simulink model "VIRTUAL_self_driving_stack_autoLocalize_v2"  (R2026a)
settings: Solver=ode1  StopTime=inf  FixedStep=1/500  EnableMultiTasking=on
values from neighbouring files (symbols this model uses):
  Controller_Sample_Time = 1/500    (= 0.002)    [Setup_QCar2_Params_Addons.m]
  path_x4 = [-0.614 -0.604 -0.594 -0.584 -0.574 -0.564 -0.554 -0.544 -0.534 -0.524 -0.514 -0.504 ... (1761 elements, 1761x1)]    [SDCS_Paths_7.mat]
  path_y4 = [-1.0887 -1.0887 -1.0887 -1.0887 -1.0887 -1.0887 -1.0887 -1.0887 -1.0887 -1.0887 -1.0887 -1.0887 ... (1761 elements, 1761x1)]    [SDCS_Paths_7.mat]
undefined symbols (not defined in the file or in its folder): AAAF5050, CSI_Sample_Time, DiscIntNeverNeededParam, gcbh, height, HIL, ImageDisplay_Sample_Time, Initialization_Time, JPEG, K12, left, LiDAR_Sample_Time, MC, qc_get_step_size, RealSense_Sample_Time, top, video_display_show, width
libraries: quarc_library x67, simulink x5, visionconversions x1, visiontransforms x1, sl_discontinuities x1
(part 1 of 3)
settings Model: ExtModeTrigDuration=10000  Creator=PKaram  LastModifiedBy=yasamin
settings SolverCC: PositivePriorityOrder=on
settings DebuggingCC: UnderspecifiedInitializationDetection=Classic  ParameterPrecisionLossMsg=none
settings SimscapeCC: SimscapeLogType=none  SimscapeNominalValues="[{\"value\":\"1\",\"unit\":\"A\"},{\"value\":\"1\",\"unit\":\"bar\"},{\"value\":\"1\",\"unit\":\"cm^2\"},{\"value\":\"1\",\"unit\":\"cm^3/s\"},{\"value\":\"1\",\"unit\":\"kJ/kg\"},{\"value\":\"1\",\"unit\":\"kW\"},{\"value\":\"1\",\"unit\":\"l\"},{\"value\":\"1\",\"unit\":\"N\"},{\"value\":\"1\",\"unit\":\"N*m\"},{\"value\":\"1\",\"unit\":\"V\"}]"  SimscapeLogDataHistory=5000.0

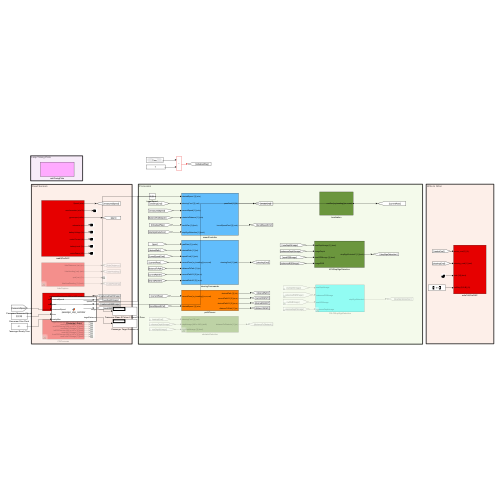
[thumbnail: Simulink's stored preview of the top-level diagram]
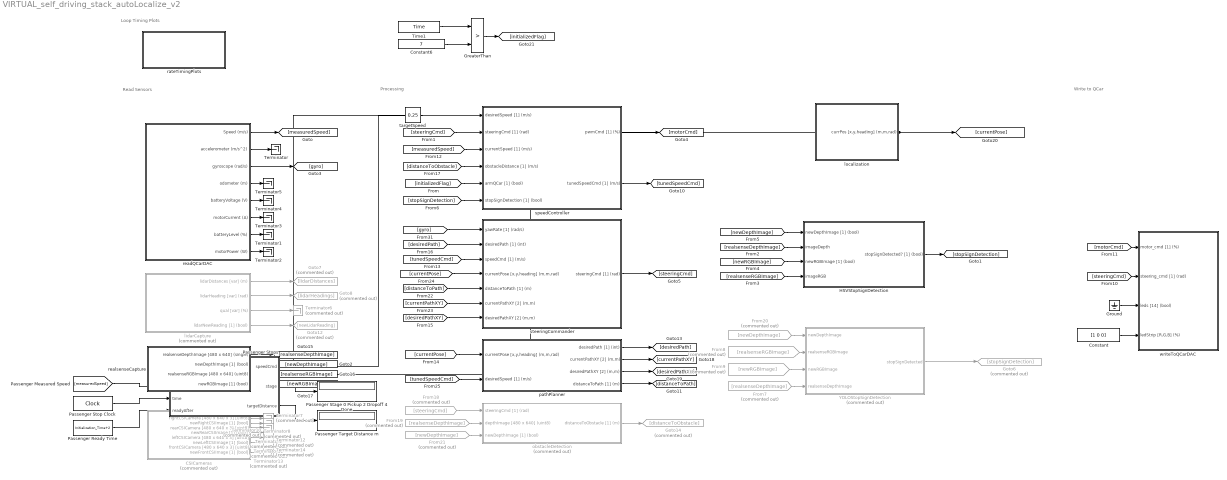
== system VIRTUAL_self_driving_stack_autoLocalize_v2 ==
  note: Loop Timing Plots
  note: Write to QCar
  note: Processing
  note: Read Sensors
  CSICameras : Subsystem  Commented=on
  Constant : Constant  Value=[1 0 0]
  Constant6 : Constant  Value=7
  From18 : From  Commented=on  GotoTag=steeringCmd
  From19 : From  Commented=on  GotoTag=realsenseDepthImage
  From20 : From  Commented=on  GotoTag=newDepthImage
  From21 : From  Commented=on  GotoTag=newDepthImage
  From7 : From  Commented=on  GotoTag=realsenseDepthImage
  From8 : From  Commented=on  GotoTag=realsenseRGBImage
  From9 : From  Commented=on  GotoTag=newRGBImage
  Goto12 : Goto  Commented=on  GotoTag=newLidarReading
  Goto14 : Goto  Commented=on  GotoTag=distanceToObstacle
  Goto6 : Goto  Commented=on  GotoTag=stopSignDetection
  Goto7 : Goto  Commented=on  GotoTag=lidarDistances
  Goto8 : Goto  Commented=on  GotoTag=lidarHeadings
  GreaterThan : RelationalOperator  Operator=>  OutDataTypeStr=boolean  RndMeth=Simplest  InputSameDT=off
  Ground : Ground
  HSVStopSignDetection : Subsystem
  Passenger Ready Time : Constant  Value=Initialization_Time+2
  Passenger Stage 0 Pickup 2 Dropoff 4 Done : Display
  Passenger Stop Clock : DigitalClock  SampleTime=Controller_Sample_Time
  Passenger Stops : MATLAB Function  TreatAsAtomicUnit=on
  Passenger Target Distance m : Display
  Terminator{,1..5} (6 alike) : Terminator
  Terminator{6..14} (9 alike) : Terminator  Commented=on
  Time1 : quarc_library/Sources/Time/Time  time_source=Wall clock  sample_time=Controller_Sample_Time
  YOLOStopSignDetection : Subsystem  Commented=on
  lidarCapture : Subsystem  Commented=on
  localization : Subsystem
  obstacleDetection : Subsystem  Commented=on
  pathPlanner : Subsystem
  rateTimingPlots : Subsystem
  readQCarDAC : Subsystem
  realsenseCapture : Subsystem
  speedController : Subsystem
  steeringCommander : Subsystem
  targetSpeed : Constant  Value=0.25
  writeToQCarDAC : Subsystem
  wires:
  readQCarDAC/6(motorCurrent (A)) -> Terminator3/1
  [tunedSpeedCmd] -> steeringCommander/3(speedCmd [1] (m/s))
  Constant/1 -> writeToQCarDAC/4(ledStrip [R,G,B] (%))
  pathPlanner/2(currentPathXY [2] (m,m)) -> [currentPathXY]
  lidarCapture/2(lidarHeading [var] (rad)) -> Goto8/1
  readQCarDAC/2(accelerometer (m/s^2)) -> Terminator/1
  Ground/1 -> writeToQCarDAC/3(leds [14] (bool))
  realsenseCapture/1(realsenseDepthImage [480 x 640] (single)) -> [realsenseDepthImage]
  [steeringCmd] -> writeToQCarDAC/2(steering_cmd [1] (rad))
  pathPlanner/4(distanceToPath [1] (m)) -> [distanceToPath]
  lidarCapture/1(lidarDistances [var] (m)) -> Goto7/1
  readQCarDAC/4(odometer (m)) -> Terminator5/1
  readQCarDAC/3(gyroscope (rad/s)) -> [gyro]
  pathPlanner/3(desiredPathXY [2] (m,m)) -> [desiredPathXY]
  From21/1 -> obstacleDetection/3(newDepthImage [1] (bool))
  [tunedSpeedCmd] -> pathPlanner/2(desiredSpeed [1] (m/s))
  readQCarDAC/5(batteryVoltage (V)) -> Terminator4/1
  readQCarDAC/1(Speed (m/s)) -> [measuredSpeed]
  speedController/2(tunedSpeedCmd [1] (m/s)) -> [tunedSpeedCmd]
  [distanceToObstacle] -> speedController/4(obstacleDistance [1] (m/s))
  [currentPathXY] -> steeringCommander/6(currentPathXY [2] (m,m))
  From19/1 -> obstacleDetection/2(depthImage [480 x 640] (uint8))
  readQCarDAC/8(motorPower (W)) -> Terminator2/1
  speedController/1(pwmCmd [1] (%)) -> [motorCmd]
  [initializedFlag] -> speedController/5(armQCar [1] (bool))
  [motorCmd] -> writeToQCarDAC/1(motor_cmd [1] (%))
  [steeringCmd] -> speedController/2(steeringCmd [1] (rad))
  lidarCapture/4(lidarNewReading [1] (bool)) -> Goto12/1
  [desiredPathXY] -> steeringCommander/7(desiredPathXY [2] (m,m))
  [distanceToPath] -> steeringCommander/5(distanceToPath [1] (m))
  realsenseCapture/4(newRGBImage [1] (bool)) -> [newRGBImage]
  lidarCapture/3(qual [var] (%)) -> Terminator6/1
  readQCarDAC/7(batteryLevel (%)) -> Terminator1/1
  [desiredPath] -> steeringCommander/2(desiredPath [1] (int))
  From18/1 -> obstacleDetection/1(steeringCmd [1] (rad))
  obstacleDetection/1(distanceToObstacle [1] (m)) -> Goto14/1
  [measuredSpeed] -> speedController/3(currentSpeed [1] (m/s))
  pathPlanner/1(desiredPath [1] (int)) -> [desiredPath]
  realsenseCapture/2(newDepthImage [1] (bool)) -> [newDepthImage]
  realsenseCapture/3("realsenseRGBImage [480 x 640] (uint8) ") -> [realsenseRGBImage]
  [currentPose] -> pathPlanner/1(currentPose [x,y,heading] (m,m,rad))
  [currentPose] -> steeringCommander/4(currentPose [x,y,heading] (m,m,rad))
  steeringCommander/1(steeringCmd [1] (rad)) -> [steeringCmd]
  [gyro] -> steeringCommander/1(yawRate [1] (rad/s))
  CSICameras/1(rightCSICamera [480 x 640 x 3] [uint8]) -> Terminator7/1
  CSICameras/2(newRightCSIImage [1] [bool]) -> Terminator8/1
  CSICameras/3(rearCSICamera [480 x 640 x 3] [uint8]) -> Terminator9/1
  CSICameras/4(newRearCSIImage [1] [bool]) -> Terminator10/1
  CSICameras/5(leftCSICamera [480 x 640 x 3] [uint8]) -> Terminator11/1
  CSICameras/6(newLeftCSIImage [1] [bool]) -> Terminator12/1
  CSICameras/7(frontCSICamera [480 x 640 x 3] [uint8]) -> Terminator13/1
  CSICameras/8(newFrontCSIImage [1] [bool]) -> Terminator14/1
  localization/1("currPos [x,y,heading] (m,m,rad) ") -> [currentPose], Passenger Stops/2(pose)
  Constant6/1 -> GreaterThan/2
  GreaterThan/1 -> [initializedFlag]
  Time1/1 -> GreaterThan/1
  [stopSignDetection] -> speedController/6(stopSignDetection [1] (bool))
  [newDepthImage] -> HSVStopSignDetection/1(newDepthImage [1] (bool))
  [realsenseDepthImage] -> HSVStopSignDetection/2(imageDepth)
  [newRGBImage] -> HSVStopSignDetection/3(newRGBImage [1] (bool))
  [realsenseRGBImage] -> HSVStopSignDetection/4(imageRGB)
  HSVStopSignDetection/1(stopSignDetected? [1] (bool)) -> [stopSignDetection]
  From20/1 -> YOLOStopSignDetection/1(newDepthImage)
  From7/1 -> YOLOStopSignDetection/4(realsenseDepthImage)
  From9/1 -> YOLOStopSignDetection/3(newRGBImage)
  YOLOStopSignDetection/1(stopSignDetected) -> Goto6/1
  From8/1 -> YOLOStopSignDetection/2(realsenseRGBImage)
  targetSpeed/1 -> Passenger Stops/1(nominalSpeed)
  [measuredSpeed] -> Passenger Stops/3(measuredSpeed)
  Passenger Stop Clock/1 -> Passenger Stops/4(time)
  Passenger Ready Time/1 -> Passenger Stops/5(readyAfter)
  Passenger Stops/1(speedCmd) -> speedController/1(desiredSpeed [1] (m/s))
  Passenger Stops/2(stage) -> Passenger Stage 0 Pickup 2 Dropoff 4 Done/1
  Passenger Stops/3(targetDistance) -> Passenger Target Distance m/1

== system VIRTUAL_self_driving_stack_autoLocalize_v2/CSICameras ==
  Video Compressed Display : Subsystem  Commented=on  LoadFcn=set_param(gcbh, 'UserData', gcb);  StartFcn=video_display_show([gcb, '/Video Display'], 'add', gcb);  mask(Video Compressed Display){algorithm=JPEG, quality=50, sample_time=-1, use_hardware=on}
      mask prompts: algorithm "Compression algorithm:"; quality "Compression quality (0-100):"; sample_time "Sample time (seconds):"; use_hardware "Use hardware acceleration for video display"
      mask help: Displays a video stream on the host, using compression to minimize bandwidth.
      mask init:
      | qc_set_display('Video\nCompressed\nDisplay');
      settings: UndoDeleteFcn=set_param(gcbh, 'UserData', gcb);  OpenFcn=video_display_show([gcb, '/Video Display'], 'show', gcb);  PreDeleteFcn=video_display_show([gcb, '/Video Display'], 'delete');
      settings: CopyFcn=|
      | set_param(gcbh, 'UserData', gcb);
      | set_param(gcbh, 'LinkStatus', 'none');
      settings: NameChangeFcn=|
      | video_display_show([get_param(gcbh, 'UserData'), '/Video Display'], 'rename', [gcb, '/Video Display']);
      | video_display_show([gcb, '/Video Display'], 'add', gcb);
      | set_param(gcbh, 'UserData', gcb);
      mask Help: web(qc_get_block_help_path(gcb));
      mask TypeOptions algorithm: Image Compress/algorithm
      mask TypeOptions quality: Image Compress/quality
      mask TypeOptions sample_time: Video Display/sample_time
      mask TypeOptions use_hardware: Video Display/use_hardware
      mask Display:
      | patch([0.98591 0.98591 0.62618 0.59072 0.56147   0.536   0.536  0.5441 0.56912 0.59207 0.60881 0.62276 0.63527 0.64364  0.6485  0.6485 0.64706 0.64499 0.63662 0.62411 0.61232 0.59837 0.58307 0.56147   0.536   0.536  0.5441  0.5747 0.60953 0.63662 0.67001  0.7034 0.72851 0.75425 0.77927 0.80294 0.82454 0.84119 0.85865 0.87395 0.88574 0.89339  0.8969 0.89969 0.89969 0.89267  0.8816 0.87044 0.85649  0.8384 0.81824 0.80294 0.78764 0.77513 0.76676 0.75776 0.76397 0.77513 0.79178 0.80987 0.82796 0.84326 0.86207 0.98528],[0.18689 0.05522 0.05522 0.05171 0.05171    0.05 0.18338 0.18338 0.19148 0.20435 0.22298 0.24863 0.28589 0.33125 0.38138 0.55139 0.59801 0.63761 0.68189 0.72149 0.74939 0.76694 0.77855 0.79367 0.79952 0.92768 0.92768 0.92768 0.92417 0.92066 0.91364  0.9032 0.89384 0.88106 0.86594 0.85073 0.82634 0.80537 0.77855 0.74363 0.70403 0.65858 0.61079 0.59099 0.41513 0.37202 0.31847 0.29048 0.25556 0.23342  0.2102 0.19382 0.18221 0.17285 0.16943 0.16124  0.1589 0.16241 0.16709 0.17168  0.1787 0.18221 0.18689 0.18689],[0.9,0.90,0.91])
      | patch([0.536 0.52601 0.46823 0.44528 0.41603 0.39101 0.35555 0.33116 0.31451 0.29291  0.2804 0.26717 0.25322 0.23999 0.22406 0.20732 0.19337 0.17528 0.15935 0.14396 0.13217 0.11759 0.10922 0.10085 0.09671 0.09392 0.09041 0.08906 0.08906 0.09464  0.0995 0.10778 0.11894 0.13145 0.14675 0.16349 0.17672 0.19409 0.20732 0.22406 0.23999 0.26159 0.27833 0.29849 0.31793 0.33602 0.35411 0.37085 0.39245 0.41603   0.536   0.536 0.53159 0.46409   0.446 0.42026 0.39587 0.37571 0.36113 0.34925 0.34088 0.33809 0.33809 0.34088 0.34583 0.35627 0.36392 0.38129 0.39587 0.41117 0.42719 0.44672  0.4676 0.48353 0.48353 0.52394   0.536],[0.05 0.04829 0.04712 0.04712 0.04829 0.05063 0.05405 0.05873 0.06107 0.06692 0.07043 0.07619 0.08087 0.08672 0.09482 0.10652 0.11696 0.13325  0.1508 0.17168 0.19499 0.22415 0.25439 0.28472 0.31379 0.35456 0.38489 0.41513 0.58055 0.63878 0.68774 0.72149 0.75641 0.78089 0.80537 0.82859 0.84029 0.85658 0.86594 0.87404  0.8834 0.89267 0.90086 0.90788 0.91247 0.91832 0.92066   0.923 0.92651 0.92768 0.92768 0.79952 0.79952 0.79952 0.79718 0.78899 0.77153 0.75056 0.72149 0.68072 0.62249  0.5549 0.41396 0.37085 0.33242 0.28121 0.25205 0.22181 0.20552 0.19499 0.18572 0.18221 0.17753 0.17636 0.17753  0.1787  0.1787],[0.9,0.90,0.91])
      | disp('Video\nCompressed\nDisplay');
  Video Compressed Display1 : Subsystem  Commented=on  LoadFcn=set_param(gcbh, 'UserData', gcb);  StartFcn=video_display_show([gcb, '/Video Display'], 'add', gcb);  mask(Video Compressed Display){algorithm=JPEG, quality=50, sample_time=-1, use_hardware=on}
      mask prompts: algorithm "Compression algorithm:"; quality "Compression quality (0-100):"; sample_time "Sample time (seconds):"; use_hardware "Use hardware acceleration for video display"
      mask help: Displays a video stream on the host, using compression to minimize bandwidth.
      mask init:
      | qc_set_display('Video\nCompressed\nDisplay');
      settings: UndoDeleteFcn=set_param(gcbh, 'UserData', gcb);  OpenFcn=video_display_show([gcb, '/Video Display'], 'show', gcb);  PreDeleteFcn=video_display_show([gcb, '/Video Display'], 'delete');
      settings: CopyFcn=|
      | set_param(gcbh, 'UserData', gcb);
      | set_param(gcbh, 'LinkStatus', 'none');
      settings: NameChangeFcn=|
      | video_display_show([get_param(gcbh, 'UserData'), '/Video Display'], 'rename', [gcb, '/Video Display']);
      | video_display_show([gcb, '/Video Display'], 'add', gcb);
      | set_param(gcbh, 'UserData', gcb);
      mask Help: web(qc_get_block_help_path(gcb));
      mask TypeOptions algorithm: Image Compress/algorithm
      mask TypeOptions quality: Image Compress/quality
      mask TypeOptions sample_time: Video Display/sample_time
      mask TypeOptions use_hardware: Video Display/use_hardware
      mask Display:
      | patch([0.98591 0.98591 0.62618 0.59072 0.56147   0.536   0.536  0.5441 0.56912 0.59207 0.60881 0.62276 0.63527 0.64364  0.6485  0.6485 0.64706 0.64499 0.63662 0.62411 0.61232 0.59837 0.58307 0.56147   0.536   0.536  0.5441  0.5747 0.60953 0.63662 0.67001  0.7034 0.72851 0.75425 0.77927 0.80294 0.82454 0.84119 0.85865 0.87395 0.88574 0.89339  0.8969 0.89969 0.89969 0.89267  0.8816 0.87044 0.85649  0.8384 0.81824 0.80294 0.78764 0.77513 0.76676 0.75776 0.76397 0.77513 0.79178 0.80987 0.82796 0.84326 0.86207 0.98528],[0.18689 0.05522 0.05522 0.05171 0.05171    0.05 0.18338 0.18338 0.19148 0.20435 0.22298 0.24863 0.28589 0.33125 0.38138 0.55139 0.59801 0.63761 0.68189 0.72149 0.74939 0.76694 0.77855 0.79367 0.79952 0.92768 0.92768 0.92768 0.92417 0.92066 0.91364  0.9032 0.89384 0.88106 0.86594 0.85073 0.82634 0.80537 0.77855 0.74363 0.70403 0.65858 0.61079 0.59099 0.41513 0.37202 0.31847 0.29048 0.25556 0.23342  0.2102 0.19382 0.18221 0.17285 0.16943 0.16124  0.1589 0.16241 0.16709 0.17168  0.1787 0.18221 0.18689 0.18689],[0.9,0.90,0.91])
      | patch([0.536 0.52601 0.46823 0.44528 0.41603 0.39101 0.35555 0.33116 0.31451 0.29291  0.2804 0.26717 0.25322 0.23999 0.22406 0.20732 0.19337 0.17528 0.15935 0.14396 0.13217 0.11759 0.10922 0.10085 0.09671 0.09392 0.09041 0.08906 0.08906 0.09464  0.0995 0.10778 0.11894 0.13145 0.14675 0.16349 0.17672 0.19409 0.20732 0.22406 0.23999 0.26159 0.27833 0.29849 0.31793 0.33602 0.35411 0.37085 0.39245 0.41603   0.536   0.536 0.53159 0.46409   0.446 0.42026 0.39587 0.37571 0.36113 0.34925 0.34088 0.33809 0.33809 0.34088 0.34583 0.35627 0.36392 0.38129 0.39587 0.41117 0.42719 0.44672  0.4676 0.48353 0.48353 0.52394   0.536],[0.05 0.04829 0.04712 0.04712 0.04829 0.05063 0.05405 0.05873 0.06107 0.06692 0.07043 0.07619 0.08087 0.08672 0.09482 0.10652 0.11696 0.13325  0.1508 0.17168 0.19499 0.22415 0.25439 0.28472 0.31379 0.35456 0.38489 0.41513 0.58055 0.63878 0.68774 0.72149 0.75641 0.78089 0.80537 0.82859 0.84029 0.85658 0.86594 0.87404  0.8834 0.89267 0.90086 0.90788 0.91247 0.91832 0.92066   0.923 0.92651 0.92768 0.92768 0.79952 0.79952 0.79952 0.79718 0.78899 0.77153 0.75056 0.72149 0.68072 0.62249  0.5549 0.41396 0.37085 0.33242 0.28121 0.25205 0.22181 0.20552 0.19499 0.18572 0.18221 0.17753 0.17636 0.17753  0.1787  0.1787],[0.9,0.90,0.91])
      | disp('Video\nCompressed\nDisplay');
  Video Compressed Display2 : Subsystem  Commented=on  LoadFcn=set_param(gcbh, 'UserData', gcb);  StartFcn=video_display_show([gcb, '/Video Display'], 'add', gcb);  mask(Video Compressed Display){algorithm=JPEG, quality=50, sample_time=-1, use_hardware=on}
      mask prompts: algorithm "Compression algorithm:"; quality "Compression quality (0-100):"; sample_time "Sample time (seconds):"; use_hardware "Use hardware acceleration for video display"
      mask help: Displays a video stream on the host, using compression to minimize bandwidth.
      mask init:
      | qc_set_display('Video\nCompressed\nDisplay');
      settings: UndoDeleteFcn=set_param(gcbh, 'UserData', gcb);  OpenFcn=video_display_show([gcb, '/Video Display'], 'show', gcb);  PreDeleteFcn=video_display_show([gcb, '/Video Display'], 'delete');
      settings: CopyFcn=|
      | set_param(gcbh, 'UserData', gcb);
      | set_param(gcbh, 'LinkStatus', 'none');
      settings: NameChangeFcn=|
      | video_display_show([get_param(gcbh, 'UserData'), '/Video Display'], 'rename', [gcb, '/Video Display']);
      | video_display_show([gcb, '/Video Display'], 'add', gcb);
      | set_param(gcbh, 'UserData', gcb);
      mask Help: web(qc_get_block_help_path(gcb));
      mask TypeOptions algorithm: Image Compress/algorithm
      mask TypeOptions quality: Image Compress/quality
      mask TypeOptions sample_time: Video Display/sample_time
      mask TypeOptions use_hardware: Video Display/use_hardware
      mask Display:
      | patch([0.98591 0.98591 0.62618 0.59072 0.56147   0.536   0.536  0.5441 0.56912 0.59207 0.60881 0.62276 0.63527 0.64364  0.6485  0.6485 0.64706 0.64499 0.63662 0.62411 0.61232 0.59837 0.58307 0.56147   0.536   0.536  0.5441  0.5747 0.60953 0.63662 0.67001  0.7034 0.72851 0.75425 0.77927 0.80294 0.82454 0.84119 0.85865 0.87395 0.88574 0.89339  0.8969 0.89969 0.89969 0.89267  0.8816 0.87044 0.85649  0.8384 0.81824 0.80294 0.78764 0.77513 0.76676 0.75776 0.76397 0.77513 0.79178 0.80987 0.82796 0.84326 0.86207 0.98528],[0.18689 0.05522 0.05522 0.05171 0.05171    0.05 0.18338 0.18338 0.19148 0.20435 0.22298 0.24863 0.28589 0.33125 0.38138 0.55139 0.59801 0.63761 0.68189 0.72149 0.74939 0.76694 0.77855 0.79367 0.79952 0.92768 0.92768 0.92768 0.92417 0.92066 0.91364  0.9032 0.89384 0.88106 0.86594 0.85073 0.82634 0.80537 0.77855 0.74363 0.70403 0.65858 0.61079 0.59099 0.41513 0.37202 0.31847 0.29048 0.25556 0.23342  0.2102 0.19382 0.18221 0.17285 0.16943 0.16124  0.1589 0.16241 0.16709 0.17168  0.1787 0.18221 0.18689 0.18689],[0.9,0.90,0.91])
      | patch([0.536 0.52601 0.46823 0.44528 0.41603 0.39101 0.35555 0.33116 0.31451 0.29291  0.2804 0.26717 0.25322 0.23999 0.22406 0.20732 0.19337 0.17528 0.15935 0.14396 0.13217 0.11759 0.10922 0.10085 0.09671 0.09392 0.09041 0.08906 0.08906 0.09464  0.0995 0.10778 0.11894 0.13145 0.14675 0.16349 0.17672 0.19409 0.20732 0.22406 0.23999 0.26159 0.27833 0.29849 0.31793 0.33602 0.35411 0.37085 0.39245 0.41603   0.536   0.536 0.53159 0.46409   0.446 0.42026 0.39587 0.37571 0.36113 0.34925 0.34088 0.33809 0.33809 0.34088 0.34583 0.35627 0.36392 0.38129 0.39587 0.41117 0.42719 0.44672  0.4676 0.48353 0.48353 0.52394   0.536],[0.05 0.04829 0.04712 0.04712 0.04829 0.05063 0.05405 0.05873 0.06107 0.06692 0.07043 0.07619 0.08087 0.08672 0.09482 0.10652 0.11696 0.13325  0.1508 0.17168 0.19499 0.22415 0.25439 0.28472 0.31379 0.35456 0.38489 0.41513 0.58055 0.63878 0.68774 0.72149 0.75641 0.78089 0.80537 0.82859 0.84029 0.85658 0.86594 0.87404  0.8834 0.89267 0.90086 0.90788 0.91247 0.91832 0.92066   0.923 0.92651 0.92768 0.92768 0.79952 0.79952 0.79952 0.79718 0.78899 0.77153 0.75056 0.72149 0.68072 0.62249  0.5549 0.41396 0.37085 0.33242 0.28121 0.25205 0.22181 0.20552 0.19499 0.18572 0.18221 0.17753 0.17636 0.17753  0.1787  0.1787],[0.9,0.90,0.91])
      | disp('Video\nCompressed\nDisplay');
  Video Compressed Display3 : Subsystem  LoadFcn=set_param(gcbh, 'UserData', gcb);  StartFcn=video_display_show([gcb, '/Video Display'], 'add', gcb);  mask(Video Compressed Display){algorithm=JPEG, quality=50, sample_time=-1, use_hardware=on}
      mask prompts: algorithm "Compression algorithm:"; quality "Compression quality (0-100):"; sample_time "Sample time (seconds):"; use_hardware "Use hardware acceleration for video display"
      mask help: Displays a video stream on the host, using compression to minimize bandwidth.
      mask init:
      | qc_set_display('Video\nCompressed\nDisplay');
      settings: UndoDeleteFcn=set_param(gcbh, 'UserData', gcb);  OpenFcn=video_display_show([gcb, '/Video Display'], 'show', gcb);  PreDeleteFcn=video_display_show([gcb, '/Video Display'], 'delete');
      settings: CopyFcn=|
      | set_param(gcbh, 'UserData', gcb);
      | set_param(gcbh, 'LinkStatus', 'none');
      settings: NameChangeFcn=|
      | video_display_show([get_param(gcbh, 'UserData'), '/Video Display'], 'rename', [gcb, '/Video Display']);
      | video_display_show([gcb, '/Video Display'], 'add', gcb);
      | set_param(gcbh, 'UserData', gcb);
      mask Help: web(qc_get_block_help_path(gcb));
      mask TypeOptions algorithm: Image Compress/algorithm
      mask TypeOptions quality: Image Compress/quality
      mask TypeOptions sample_time: Video Display/sample_time
      mask TypeOptions use_hardware: Video Display/use_hardware
      mask Display:
      | patch([0.98591 0.98591 0.62618 0.59072 0.56147   0.536   0.536  0.5441 0.56912 0.59207 0.60881 0.62276 0.63527 0.64364  0.6485  0.6485 0.64706 0.64499 0.63662 0.62411 0.61232 0.59837 0.58307 0.56147   0.536   0.536  0.5441  0.5747 0.60953 0.63662 0.67001  0.7034 0.72851 0.75425 0.77927 0.80294 0.82454 0.84119 0.85865 0.87395 0.88574 0.89339  0.8969 0.89969 0.89969 0.89267  0.8816 0.87044 0.85649  0.8384 0.81824 0.80294 0.78764 0.77513 0.76676 0.75776 0.76397 0.77513 0.79178 0.80987 0.82796 0.84326 0.86207 0.98528],[0.18689 0.05522 0.05522 0.05171 0.05171    0.05 0.18338 0.18338 0.19148 0.20435 0.22298 0.24863 0.28589 0.33125 0.38138 0.55139 0.59801 0.63761 0.68189 0.72149 0.74939 0.76694 0.77855 0.79367 0.79952 0.92768 0.92768 0.92768 0.92417 0.92066 0.91364  0.9032 0.89384 0.88106 0.86594 0.85073 0.82634 0.80537 0.77855 0.74363 0.70403 0.65858 0.61079 0.59099 0.41513 0.37202 0.31847 0.29048 0.25556 0.23342  0.2102 0.19382 0.18221 0.17285 0.16943 0.16124  0.1589 0.16241 0.16709 0.17168  0.1787 0.18221 0.18689 0.18689],[0.9,0.90,0.91])
      | patch([0.536 0.52601 0.46823 0.44528 0.41603 0.39101 0.35555 0.33116 0.31451 0.29291  0.2804 0.26717 0.25322 0.23999 0.22406 0.20732 0.19337 0.17528 0.15935 0.14396 0.13217 0.11759 0.10922 0.10085 0.09671 0.09392 0.09041 0.08906 0.08906 0.09464  0.0995 0.10778 0.11894 0.13145 0.14675 0.16349 0.17672 0.19409 0.20732 0.22406 0.23999 0.26159 0.27833 0.29849 0.31793 0.33602 0.35411 0.37085 0.39245 0.41603   0.536   0.536 0.53159 0.46409   0.446 0.42026 0.39587 0.37571 0.36113 0.34925 0.34088 0.33809 0.33809 0.34088 0.34583 0.35627 0.36392 0.38129 0.39587 0.41117 0.42719 0.44672  0.4676 0.48353 0.48353 0.52394   0.536],[0.05 0.04829 0.04712 0.04712 0.04829 0.05063 0.05405 0.05873 0.06107 0.06692 0.07043 0.07619 0.08087 0.08672 0.09482 0.10652 0.11696 0.13325  0.1508 0.17168 0.19499 0.22415 0.25439 0.28472 0.31379 0.35456 0.38489 0.41513 0.58055 0.63878 0.68774 0.72149 0.75641 0.78089 0.80537 0.82859 0.84029 0.85658 0.86594 0.87404  0.8834 0.89267 0.90086 0.90788 0.91247 0.91832 0.92066   0.923 0.92651 0.92768 0.92768 0.79952 0.79952 0.79952 0.79718 0.78899 0.77153 0.75056 0.72149 0.68072 0.62249  0.5549 0.41396 0.37085 0.33242 0.28121 0.25205 0.22181 0.20552 0.19499 0.18572 0.18221 0.17753 0.17636 0.17753  0.1787  0.1787],[0.9,0.90,0.91])
      | disp('Video\nCompressed\nDisplay');
  frontCSICamera : quarc_library/Multimedia/Video Capture  source=device  device=3@tcpip://localhost:18964  filename=sample_movie.mov  value=[0 0; 0 0]  resolution=640 x 480  width=640  height=480  output_format=MATLAB RGB (HxWx3)  data_type=uint8  sample_time=CSI_Sample_Time  brightness_override=Do not override  brightness=50.0  contrast_override=Do not override  contrast=50.0  hue_override=Do not override  hue=50.0  saturation_override=Do not override  saturation=50.0  sharpness_override=Do not override  sharpness=50.0  gamma_override=Do not override  gamma=50.0  coloreffect_override=Do not override  coloreffect=None  whitebalance_override=Do not override  whitebalance=50.0  backlightcompensation_override=Do not override  backlightcompensation=0.0  gain_override=Do not override  gain=50.0  pan_override=Do not override  pan=50.0  tilt_override=Do not override  tilt=50.0  roll_override=Do not override  roll=50.0  zoom_override=Do not override  zoom=0.0  exposure_override=Do not override  exposure=50.0  iris_override=Do not override  iris=50.0  mirror_override=Do not override  mirror=None  focus_override=Do not override  focus=0.0
      settings: SourceProductName=QUARC Targets
  leftCSICamera : quarc_library/Multimedia/Video Capture  source=device  device=2@tcpip://localhost:18963  filename=sample_movie.mov  value=[0 0; 0 0]  resolution=640 x 480  width=640  height=480  output_format=MATLAB RGB (HxWx3)  data_type=uint8  sample_time=CSI_Sample_Time  brightness_override=Do not override  brightness=50.0  contrast_override=Do not override  contrast=50.0  hue_override=Do not override  hue=50.0  saturation_override=Do not override  saturation=50.0  sharpness_override=Do not override  sharpness=50.0  gamma_override=Do not override  gamma=50.0  coloreffect_override=Do not override  coloreffect=None  whitebalance_override=Do not override  whitebalance=50.0  backlightcompensation_override=Do not override  backlightcompensation=0.0  gain_override=Do not override  gain=50.0  pan_override=Do not override  pan=50.0  tilt_override=Do not override  tilt=50.0  roll_override=Do not override  roll=50.0  zoom_override=Do not override  zoom=0.0  exposure_override=Do not override  exposure=50.0  iris_override=Do not override  iris=50.0  mirror_override=Do not override  mirror=None  focus_override=Do not override  focus=0.0
      settings: SourceProductName=QUARC Targets
  rearCSICamera : quarc_library/Multimedia/Video Capture  source=device  device=1@tcpip://localhost:18962  filename=sample_movie.mov  value=[0 0; 0 0]  resolution=640 x 480  width=640  height=480  output_format=MATLAB RGB (HxWx3)  data_type=uint8  sample_time=CSI_Sample_Time  brightness_override=Do not override  brightness=50.0  contrast_override=Do not override  contrast=50.0  hue_override=Do not override  hue=50.0  saturation_override=Do not override  saturation=50.0  sharpness_override=Do not override  sharpness=50.0  gamma_override=Do not override  gamma=50.0  coloreffect_override=Do not override  coloreffect=None  whitebalance_override=Do not override  whitebalance=50.0  backlightcompensation_override=Do not override  backlightcompensation=0.0  gain_override=Do not override  gain=50.0  pan_override=Do not override  pan=50.0  tilt_override=Do not override  tilt=50.0  roll_override=Do not override  roll=50.0  zoom_override=Do not override  zoom=0.0  exposure_override=Do not override  exposure=50.0  iris_override=Do not override  iris=50.0  mirror_override=Do not override  mirror=None  focus_override=Do not override  focus=0.0
      settings: SourceProductName=QUARC Targets
  rightCSICamera : quarc_library/Multimedia/Video Capture  source=device  device=0@tcpip://localhost:18961  filename=sample_movie.mov  value=[0 0; 0 0]  resolution=640 x 480  width=640  height=480  output_format=MATLAB RGB (HxWx3)  data_type=uint8  sample_time=CSI_Sample_Time  brightness_override=Do not override  brightness=50.0  contrast_override=Do not override  contrast=50.0  hue_override=Do not override  hue=50.0  saturation_override=Do not override  saturation=50.0  sharpness_override=Do not override  sharpness=50.0  gamma_override=Do not override  gamma=50.0  coloreffect_override=Do not override  coloreffect=None  whitebalance_override=Do not override  whitebalance=50.0  backlightcompensation_override=Do not override  backlightcompensation=0.0  gain_override=Do not override  gain=50.0  pan_override=Do not override  pan=50.0  tilt_override=Do not override  tilt=50.0  roll_override=Do not override  roll=50.0  zoom_override=Do not override  zoom=0.0  exposure_override=Do not override  exposure=50.0  iris_override=Do not override  iris=50.0  mirror_override=Do not override  mirror=None  focus_override=Do not override  focus=0.0
      settings: SourceProductName=QUARC Targets
  rightCSICamera [480 x 640 x 3] [uint8] : Outport
  newRightCSIImage [1] [bool] : Outport  Port=2
  rearCSICamera [480 x 640 x 3] [uint8] : Outport  Port=3  VectorParamsAs1DForOutWhenUnconnected=off
  newRearCSIImage [1] [bool] : Outport  Port=4  VectorParamsAs1DForOutWhenUnconnected=off
  leftCSICamera [480 x 640 x 3] [uint8] : Outport  Port=5  VectorParamsAs1DForOutWhenUnconnected=off
  newLeftCSIImage [1] [bool] : Outport  Port=6  VectorParamsAs1DForOutWhenUnconnected=off
  frontCSICamera [480 x 640 x 3] [uint8] : Outport  Port=7  VectorParamsAs1DForOutWhenUnconnected=off
  newFrontCSIImage [1] [bool] : Outport  Port=8  VectorParamsAs1DForOutWhenUnconnected=off
  wires:
  rightCSICamera/2 -> newRightCSIImage [1] [bool]/1
  rightCSICamera/1 -> Video Compressed Display/1(In1), rightCSICamera [480 x 640 x 3] [uint8]/1
  rearCSICamera/2 -> newRearCSIImage [1] [bool]/1
  rearCSICamera/1 -> Video Compressed Display1/1(In1), rearCSICamera [480 x 640 x 3] [uint8]/1
  leftCSICamera/1 -> Video Compressed Display2/1(In1), leftCSICamera [480 x 640 x 3] [uint8]/1
  leftCSICamera/2 -> newLeftCSIImage [1] [bool]/1
  frontCSICamera/1 -> Video Compressed Display3/1(In1), frontCSICamera [480 x 640 x 3] [uint8]/1
  frontCSICamera/2 -> newFrontCSIImage [1] [bool]/1

== system VIRTUAL_self_driving_stack_autoLocalize_v2/HSVStopSignDetection ==
  newDepthImage [1] (bool) : Inport
  imageDepth : Inport  Port=2
  newRGBImage [1] (bool) : Inport  Port=3
  imageRGB : Inport  Port=4
  Compare To Constant : simulink/Logic and Bit Operations/Compare To Constant  relop=<=  const=1.2  OutDataTypeStr=boolean
  Display1 : Display
  Logical Operator : Logic  AllPortsSameDT=off  OutDataTypeStr=boolean
  findStopSignDistance : Subsystem
  findStopSignLocation : Subsystem
  stopSignDetected? [1] (bool) : Outport
  wires:
  findStopSignLocation/1(blobFound?) -> Logical Operator/2
  findStopSignDistance/1(distanceToSign (m)) -> Display1/1, Compare To Constant/1
  findStopSignLocation/2(blobLocation (px) [2]) -> findStopSignDistance/2(blobCenter (px) [2])
  Logical Operator/1 -> findStopSignDistance/Enable
  Compare To Constant/1 -> stopSignDetected? [1] (bool)/1, [stopSignDetection]
  newRGBImage [1] (bool)/1 -> findStopSignLocation/Enable
  newDepthImage [1] (bool)/1 -> Logical Operator/1
  imageDepth/1 -> findStopSignDistance/1(imageDepth)
  imageRGB/1 -> findStopSignLocation/1(imageRGB)

== system VIRTUAL_self_driving_stack_autoLocalize_v2/YOLOStopSignDetection ==
  note: Stop sign detection pre-process
  note: Video Outputs
  note: Stop sign,lane line, stop line with YOLO
  newDepthImage : Inport
  realsenseRGBImage : Inport  Port=2
  newRGBImage : Inport  Port=3
  realsenseDepthImage : Inport  Port=4
  Display : Display
  Edge Detection : Subsystem
  Four Tile Video Viewer : MATLABSystem  Commented=on  System=FourTileVideoViewer  ShowWindow=true  CloseOnRelease=false  SimulateUsing=Interpreted execution
      mask Type: FourTileVideoViewer
  Hough Transform : Subsystem
  Subsystem : Subsystem
  stopSignDetected : Outport
  wires:
  Edge Detection/1(Out1) -> Four Tile Video Viewer/2
  Hough Transform/1(Out1) -> Four Tile Video Viewer/3
  Subsystem/4(annot output) -> Four Tile Video Viewer/4
  realsenseRGBImage/1 -> Four Tile Video Viewer/1, Subsystem/2(realsenseRGBImage), Hough Transform/1(realsenseRGBImage), Edge Detection/1(realsenseRGBImage)
  Subsystem/1(distances) -> Display/1
  realsenseDepthImage/1 -> Subsystem/1(realsenseDepthImage)

== system VIRTUAL_self_driving_stack_autoLocalize_v2/lidarCapture ==
  Ranging Sensor : quarc_library/Devices/Third-Party/Sensors/Ranging Sensor  sensor_type=RPLidar LIDAR  uri=tcpip://localhost:18966  ranging_distance=Long  timing_budget=0.033  measurement_period=0.040  output_mode=Variable-size output  samples_per_revolution=SPR_qcar2  max_distance=0.050  max_angle=5  sample_time=LiDAR_Sample_Time  show_versions=on  active=on
      settings: SourceProductName=QUARC Targets
  Terminator : Terminator
  lidarFirmwareVer : Display
      settings: Decimation=100
  lidarHardwareVer : Display
      settings: Decimation=100
  lidarModel : Display
      settings: Decimation=100
  lidarDistances [var] (m) : Outport  VectorParamsAs1DForOutWhenUnconnected=off
  lidarHeading [var] (rad) : Outport  Port=2  VectorParamsAs1DForOutWhenUnconnected=off
  qual [var] (%) : Outport  Port=3  VectorParamsAs1DForOutWhenUnconnected=off
  lidarNewReading [1] (bool) : Outport  Port=4  VectorParamsAs1DForOutWhenUnconnected=off
  wires:
  Ranging Sensor/5 -> lidarNewReading [1] (bool)/1
  Ranging Sensor/7 -> lidarHardwareVer/1
  Ranging Sensor/8 -> lidarFirmwareVer/1
  Ranging Sensor/6 -> lidarModel/1
  Ranging Sensor/4 -> qual [var] (%)/1
  Ranging Sensor/1 -> lidarDistances [var] (m)/1
  Ranging Sensor/2 -> Terminator/1
  Ranging Sensor/3 -> lidarHeading [var] (rad)/1

== system VIRTUAL_self_driving_stack_autoLocalize_v2/localization ==
  Data Type Conversion1 : DataTypeConversion  OutDataTypeStr=double  SaturateOnIntegerOverflow=off  RndMeth=Floor
  Data Type Conversion2 : DataTypeConversion  OutDataTypeStr=double  SaturateOnIntegerOverflow=off  RndMeth=Floor
  Display : Display
  Inverse Modulus : quarc_library/Discontinuities/Inverse Modulus  modulus=2*pi  output_derivative=off  output_revolutions=off  max_x=Inf  min_x=-Inf
  Mux : Mux  Inputs=2
  Selector : Selector  InputPortWidth=6  IndexOptions=Index vector (dialog)  Indices=[1 2]  OutputSizes=1
  Selector1 : Selector  InputPortWidth=6  IndexOptions=Index vector (dialog)  Indices=[6]  OutputSizes=1
  Stream Client : quarc_library/Communications/Basic/Stream Client  uri_source=Specify via dialog (do not evaluate)  uri=tcpip://localhost:18967  send_buffer_size=1460  receive_buffer_size=1460  byte_order=little endian (Intel - LSB first)  optimization=Minimum latency  send_options=Do not send data  receive_options=Receive most recent data  default_value=[0 0 0 0 0 0]  sample_time=Controller_Sample_Time  active=on  implementation=Use blocking I/O in a separate thread  send_fifo_size=1000  receive_fifo_size=1000  send_priority=0  receive_priority=0  send_dimensions=off  receive_dimensions=off  max_dimensions=-1  data_type=single  type_expr=BusObject
      settings: AttributesFormatString="\"tcpip://localhost:18967\""
  Subsystem : Subsystem
  Terminator15 : Terminator
  Terminator16 : Terminator
  "currPos [x,y,heading] (m,m,rad) " : Outport
  wires:
  Subsystem/1(Mod_Angle) -> Mux/2
  Stream Client/2 -> Terminator16/1
  Selector/1 -> Data Type Conversion2/1
  Data Type Conversion2/1 -> Mux/1
  Data Type Conversion1/1 -> Inverse Modulus/1
  Stream Client/1 -> Display/1
  Stream Client/3 -> Selector/1, Selector1/1
  Selector1/1 -> Data Type Conversion1/1
  Inverse Modulus/1 -> Subsystem/1(Angle)
  Stream Client/4 -> Terminator15/1
  Mux/1 -> "currPos [x,y,heading] (m,m,rad) "/1

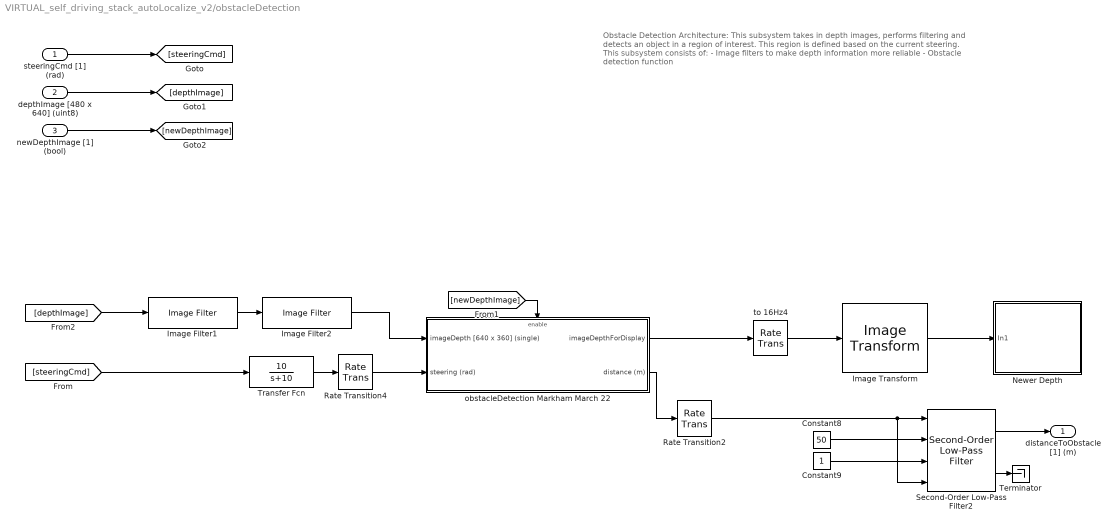
== system VIRTUAL_self_driving_stack_autoLocalize_v2/obstacleDetection ==
  note: Obstacle Detection Architecture:
      |
      | This subsystem takes in depth images, performs filtering and detects an object in a region of interest. This region is defined based on the current steering.
      |
      | This subsystem consists of:
      |
      | - Image filters to make depth information more reliable
      | - Obstacle detection function
  steeringCmd [1] (rad) : Inport
  depthImage [480 x 640] (uint8) : Inport  Port=2
  newDepthImage [1] (bool) : Inport  Port=3
  Constant8 : Constant  Value=50
  Constant9 : Constant
  Image Filter1 : quarc_library/Image Processing/Generic/Image Filter  filter_type=Depth temporal low-pass  source_of_roi=Internal dialog parameter  roi_style=[top, left, height, width]  roi=[]  maximum_roi=[]  roi_zone=Operate inside region of interest  border_type=Replicate  border_value=[0 0 0]  kernel_size=5  sigma=10  mask_size=[3 3]  kernel=int16([-2 -1 0; -1 1 1; 0 1 2])  divisor=1  offset=0  rounding=Nearest  algorithm_hint=None  threshold=1  alpha=0.9  num_frames=8  num_valid=1  gap_threshold=10  depth_threshold=255  iterations=2  norm_type=L1
      settings: AttributesFormatString=(%<filter_type>)  SourceProductName=QUARC Targets
  Image Filter2 : quarc_library/Image Processing/Generic/Image Filter  filter_type=Depth hole-fill  source_of_roi=Internal dialog parameter  roi_style=[top, left, height, width]  roi=[]  maximum_roi=[]  roi_zone=Operate inside region of interest  border_type=Replicate  border_value=[0 0 0]  kernel_size=5  sigma=10  mask_size=[3 3]  kernel=int16([-2 -1 0; -1 1 1; 0 1 2])  divisor=1  offset=0  rounding=Nearest  algorithm_hint=None  threshold=100  alpha=0.9  num_frames=8  num_valid=1  gap_threshold=10  depth_threshold=255  iterations=2  norm_type=L1
      settings: AttributesFormatString=(%<filter_type>)  SourceProductName=QUARC Targets
  Image Transform : quarc_library/Image Processing/Generic/Image Transform  algorithm=Colorize  color_theme=KRYGCBMW  min_pixel=0  max_pixel=65535  contour_depth=1  focal_length=308  principal_point=[262 334]  radial_coeffs=[-0.3129 0.0907]  tangential_coeffs=[]  extrapolated_pixel=0  interpolation=nearest  row_coords=0  column_coords=0  output_height=480  output_width=640  angle=0  origin=[240 320]  output_origin=[240 320]  output_data_type=uint8
      settings: AttributesFormatString=(%<algorithm>)  SourceProductName=QUARC Targets
  Newer Depth : Subsystem  LoadFcn=set_param(gcbh, 'UserData', gcb);  StartFcn=video_display_show([gcb, '/Video Display'], 'add', gcb);  mask(Video Compressed Display){algorithm=JPEG, quality=50, sample_time=-1, use_hardware=on}
      mask prompts: algorithm "Compression algorithm:"; quality "Compression quality (0-100):"; sample_time "Sample time (seconds):"; use_hardware "Use hardware acceleration for video display"
      mask help: Displays a video stream on the host, using compression to minimize bandwidth.
      mask init:
      | qc_set_display('Video\nCompressed\nDisplay');
      settings: UndoDeleteFcn=set_param(gcbh, 'UserData', gcb);  OpenFcn=video_display_show([gcb, '/Video Display'], 'show', gcb);  PreDeleteFcn=video_display_show([gcb, '/Video Display'], 'delete');
      settings: CopyFcn=|
      | set_param(gcbh, 'UserData', gcb);
      | set_param(gcbh, 'LinkStatus', 'none');
      settings: NameChangeFcn=|
      | video_display_show([get_param(gcbh, 'UserData'), '/Video Display'], 'rename', [gcb, '/Video Display']);
      | video_display_show([gcb, '/Video Display'], 'add', gcb);
      | set_param(gcbh, 'UserData', gcb);
      mask Help: web(qc_get_block_help_path(gcb));
      mask TypeOptions algorithm: Image Compress/algorithm
      mask TypeOptions quality: Image Compress/quality
      mask TypeOptions sample_time: Video Display/sample_time
      mask TypeOptions use_hardware: Video Display/use_hardware
      mask Display:
      | patch([0.98591 0.98591 0.62618 0.59072 0.56147   0.536   0.536  0.5441 0.56912 0.59207 0.60881 0.62276 0.63527 0.64364  0.6485  0.6485 0.64706 0.64499 0.63662 0.62411 0.61232 0.59837 0.58307 0.56147   0.536   0.536  0.5441  0.5747 0.60953 0.63662 0.67001  0.7034 0.72851 0.75425 0.77927 0.80294 0.82454 0.84119 0.85865 0.87395 0.88574 0.89339  0.8969 0.89969 0.89969 0.89267  0.8816 0.87044 0.85649  0.8384 0.81824 0.80294 0.78764 0.77513 0.76676 0.75776 0.76397 0.77513 0.79178 0.80987 0.82796 0.84326 0.86207 0.98528],[0.18689 0.05522 0.05522 0.05171 0.05171    0.05 0.18338 0.18338 0.19148 0.20435 0.22298 0.24863 0.28589 0.33125 0.38138 0.55139 0.59801 0.63761 0.68189 0.72149 0.74939 0.76694 0.77855 0.79367 0.79952 0.92768 0.92768 0.92768 0.92417 0.92066 0.91364  0.9032 0.89384 0.88106 0.86594 0.85073 0.82634 0.80537 0.77855 0.74363 0.70403 0.65858 0.61079 0.59099 0.41513 0.37202 0.31847 0.29048 0.25556 0.23342  0.2102 0.19382 0.18221 0.17285 0.16943 0.16124  0.1589 0.16241 0.16709 0.17168  0.1787 0.18221 0.18689 0.18689],[0.9,0.90,0.91])
      | patch([0.536 0.52601 0.46823 0.44528 0.41603 0.39101 0.35555 0.33116 0.31451 0.29291  0.2804 0.26717 0.25322 0.23999 0.22406 0.20732 0.19337 0.17528 0.15935 0.14396 0.13217 0.11759 0.10922 0.10085 0.09671 0.09392 0.09041 0.08906 0.08906 0.09464  0.0995 0.10778 0.11894 0.13145 0.14675 0.16349 0.17672 0.19409 0.20732 0.22406 0.23999 0.26159 0.27833 0.29849 0.31793 0.33602 0.35411 0.37085 0.39245 0.41603   0.536   0.536 0.53159 0.46409   0.446 0.42026 0.39587 0.37571 0.36113 0.34925 0.34088 0.33809 0.33809 0.34088 0.34583 0.35627 0.36392 0.38129 0.39587 0.41117 0.42719 0.44672  0.4676 0.48353 0.48353 0.52394   0.536],[0.05 0.04829 0.04712 0.04712 0.04829 0.05063 0.05405 0.05873 0.06107 0.06692 0.07043 0.07619 0.08087 0.08672 0.09482 0.10652 0.11696 0.13325  0.1508 0.17168 0.19499 0.22415 0.25439 0.28472 0.31379 0.35456 0.38489 0.41513 0.58055 0.63878 0.68774 0.72149 0.75641 0.78089 0.80537 0.82859 0.84029 0.85658 0.86594 0.87404  0.8834 0.89267 0.90086 0.90788 0.91247 0.91832 0.92066   0.923 0.92651 0.92768 0.92768 0.79952 0.79952 0.79952 0.79718 0.78899 0.77153 0.75056 0.72149 0.68072 0.62249  0.5549 0.41396 0.37085 0.33242 0.28121 0.25205 0.22181 0.20552 0.19499 0.18572 0.18221 0.17753 0.17636 0.17753  0.1787  0.1787],[0.9,0.90,0.91])
      | disp('Video\nCompressed\nDisplay');
  Rate Transition2 : RateTransition
  Rate Transition4 : RateTransition  Deterministic=off
  Second-Order Low-Pass Filter2 : quarc_library/Continuous/Second-Order Low-Pass Filter  params_source=External (input ports)  input_width=1  input_zeta=1  input_init=0
  Terminator : Terminator
  Transfer Fcn : TransferFcn  Numerator=[10]  Denominator=[1 10]
  obstacleDetection Markham March 22 : Subsystem
  to 16Hz4 : RateTransition  Deterministic=off  OutPortSampleTime=ImageDisplay_Sample_Time
  distanceToObstacle [1] (m) : Outport
  wires:
  Transfer Fcn/1 -> Rate Transition4/1
  steeringCmd [1] (rad)/1 -> [steeringCmd]
  Constant9/1 -> Second-Order Low-Pass Filter2/3
  obstacleDetection Markham March 22/2(distance (m)) -> Rate Transition2/1
  Rate Transition2/1 -> Second-Order Low-Pass Filter2/4, Second-Order Low-Pass Filter2/1
  obstacleDetection Markham March 22/1(imageDepthForDisplay) -> to 16Hz4/1
  Second-Order Low-Pass Filter2/2 -> Terminator/1
  Rate Transition4/1 -> obstacleDetection Markham March 22/2(steering (rad))
  Constant8/1 -> Second-Order Low-Pass Filter2/2
  Second-Order Low-Pass Filter2/1 -> distanceToObstacle [1] (m)/1
  to 16Hz4/1 -> Image Transform/1
  Image Transform/1 -> Newer Depth/1(In1)
  [steeringCmd] -> Transfer Fcn/1
  depthImage [480 x 640] (uint8)/1 -> [depthImage]
  newDepthImage [1] (bool)/1 -> [newDepthImage]
  [newDepthImage] -> obstacleDetection Markham March 22/Enable
  [depthImage] -> Image Filter1/1
  Image Filter1/1 -> Image Filter2/1
  Image Filter2/1 -> obstacleDetection Markham March 22/1(imageDepth [640 x 360] (single))

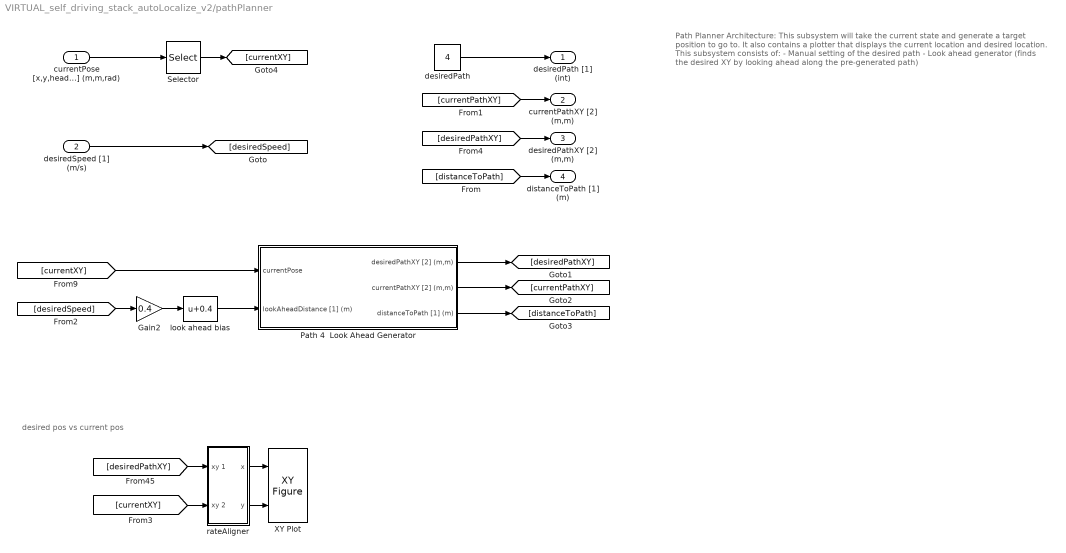
== system VIRTUAL_self_driving_stack_autoLocalize_v2/pathPlanner ==
  note: desired pos vs current pos
  note: Path Planner Architecture:
      |
      | This subsystem will take the current state and generate a target position to go to. It also contains a plotter that displays the current location and desired location.
      |
      | This subsystem consists of:
      |
      | - Manual setting of the desired path
      | - Look ahead generator (finds the desired XY by looking ahead along the pre-generated path)
  currentPose [x,y,heading] (m,m,rad) : Inport
  desiredSpeed [1] (m/s) : Inport  Port=2
  Gain2 : Gain  Gain=0.4
  Path 4  Look Ahead Generator : Subsystem
  Selector : Selector  InputPortWidth=3  IndexOptions=Index vector (dialog)  Indices=[1 2]  OutputSizes=1
  XY Plot : quarc_library/Sinks/Figures/XY Figure  figure_mode=Use figure window  figure_tag=figure1  axes_tag=axes1  plot_mode=Time-based  minimum_x=-2.5  maximum_x=2.5  minimum_y=-2  maximum_y=5  buffer_size=100  update_rate=1  initial_position="3522    50   958   817"  initial_visibility=off  sample_time=-1
      settings: SourceProductName=QUARC Targets
  desiredPath : Constant  Value=4
  look ahead bias : Bias  Bias=0.4  SaturateOnIntegerOverflow=off
  rateAligner : Subsystem
  desiredPath [1] (int) : Outport
  currentPathXY [2] (m,m) : Outport  Port=2
  desiredPathXY [2] (m,m) : Outport  Port=3
  distanceToPath [1] (m) : Outport  Port=4
  wires:
  desiredPath/1 -> desiredPath [1] (int)/1
  [desiredSpeed] -> Gain2/1
  Gain2/1 -> look ahead bias/1
  [currentXY] -> Path 4  Look Ahead Generator/1(currentPose)
  rateAligner/1(x) -> XY Plot/1
  rateAligner/2(y) -> XY Plot/2
  [desiredPathXY] -> rateAligner/1(xy 1)
  [currentXY] -> rateAligner/2(xy 2)
  currentPose [x,y,heading] (m,m,rad)/1 -> Selector/1
  desiredSpeed [1] (m/s)/1 -> [desiredSpeed]
  Path 4  Look Ahead Generator/1(desiredPathXY [2] (m,m)) -> [desiredPathXY]
  Selector/1 -> [currentXY]
  Path 4  Look Ahead Generator/2(currentPathXY [2] (m,m)) -> [currentPathXY]
  Path 4  Look Ahead Generator/3(distanceToPath [1] (m)) -> [distanceToPath]
  [distanceToPath] -> distanceToPath [1] (m)/1
  [currentPathXY] -> currentPathXY [2] (m,m)/1
  [desiredPathXY] -> desiredPathXY [2] (m,m)/1
  look ahead bias/1 -> Path 4  Look Ahead Generator/2(lookAheadDistance [1] (m))

== system VIRTUAL_self_driving_stack_autoLocalize_v2/rateTimingPlots ==
  CSI : Scope
  Control : Scope
      settings: ActiveDisplayYMinimum=-0.0041135  ActiveDisplayYMaximum=0.012664
  Image Displays : Scope
  LCD : Scope
  LiDAR : Scope
  RealSense : Scope
  monitorTiming : Subsystem
  monitorTiming1 : Subsystem
  monitorTiming2 : Subsystem
  monitorTiming3 : Subsystem
  monitorTiming5 : Subsystem
  monitorTiming7 : Subsystem
  wires:
  monitorTiming/1(Timing (s)) -> CSI/1
  monitorTiming1/1(Timing (s)) -> Control/1
  monitorTiming3/1(Timing (s)) -> Image Displays/1
  monitorTiming2/1(Timing (s)) -> RealSense/1
  monitorTiming5/1(Timing (s)) -> LiDAR/1
  monitorTiming7/1(Timing (s)) -> LCD/1
